simulink model "pid_actuator_saturation"  (R2026b)
settings: Solver=ode4  StopTime=30  FixedStep=0.05
settings Model: Creator=ZAID  LastModifiedBy=ZAID

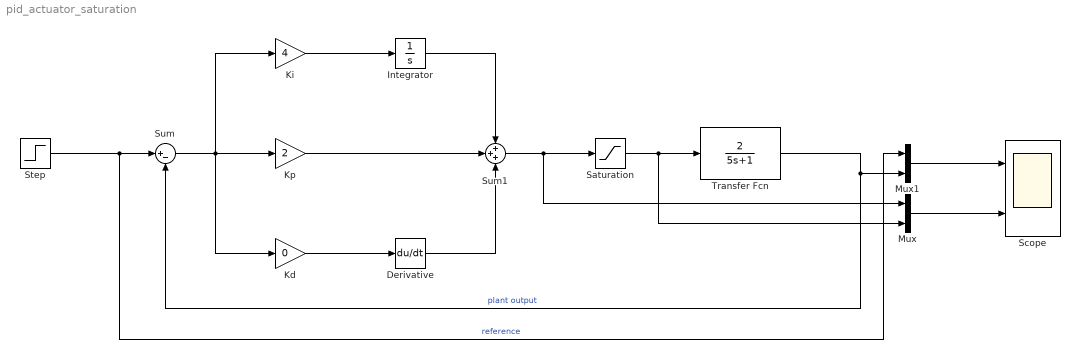
== system pid_actuator_saturation ==
  Derivative : Derivative
  Integrator : Integrator
  Kd : Gain  Gain=0
  Ki : Gain  Gain=4
  Kp : Gain  Gain=2
  Mux : Mux  Inputs=2
  Mux1 : Mux  Inputs=2
  Saturation : Saturate  UpperLimit=10  LowerLimit=-10
  Scope : Scope  NumInputPorts=2
      settings: ActiveDisplayYMinimum=-20.436598009113009  ActiveDisplayYMaximum=182.16709704513175
  Step : Step  FinalValue=15  SampleTime=0
  Sum : Sum  Inputs=|+-
  Sum1 : Sum  Inputs=+++
  Transfer Fcn : TransferFcn  Numerator=2  Denominator=[5 1]
  wires:
  Step/1 -> Mux1/1, Sum/1  "reference"
  Sum/1 -> Ki/1, Kd/1, Kp/1
  Ki/1 -> Integrator/1
  Kd/1 -> Derivative/1
  Kp/1 -> Sum1/2
  Integrator/1 -> Sum1/1
  Derivative/1 -> Sum1/3
  Sum1/1 -> Mux/1, Saturation/1
  Transfer Fcn/1 -> Mux1/2, Sum/2  "plant output"
  Saturation/1 -> Mux/2, Transfer Fcn/1
  Mux/1 -> Scope/2
  Mux1/1 -> Scope/1
